simulink model "gm_soc_dlmc_rfsoc_dut"  (R2025b)
settings: Solver=FixedStepDiscrete  StartTime=0.0  StopTime=simTime  RelTol=1e-3
PreLoadFcn:
  | addpath('E:\AMC_Projects\deployModule\AMCMatlab\hdl_prj\hdlsrc\soc_dlmc_rfsoc_zcu111');
InitFcn:
  | soc_dlmc_rfsoc_init
undefined symbols (not defined in the file or in its folder): Fo, FPGAClkRate, Fs, mcTestData8PSK, mcTestDataB_FM, mcTestDataBPSK, mcTestDataCPFSK, mcTestDataDSB_AM, mcTestDataGFSK, mcTestDataPAM4, mcTestDataQAM16, mcTestDataQAM64, mcTestDataQPSK, mcTestDataSSB_AM, N, sampleTimeDL
libraries: hdlsllib x15, hdlmdlgenlib x9, simulink x2, simulink_need_slupdate x2, dsphdlsigops2 x1
CloseFcn:
  | addpath('E:\AMC_Projects\deployModule\AMCMatlab\hdl_prj\hdlsrc\soc_dlmc_rfsoc_zcu111');
  | rmpath('E:\AMC_Projects\deployModule\AMCMatlab\hdl_prj\hdlsrc\soc_dlmc_rfsoc_zcu111');
settings Model: Creator=The MathWorks, Inc.  LastModifiedBy=admin
settings SolverCC: AlgebraicLoopSolver=TrustRegion  PositivePriorityOrder=on  MaxZcPerStep=1.0
settings DataIOCC: SaveOutput=off  SaveTime=off
settings OptimizationCC: BlockReduction=off  ConditionallyExecuteInputs=off  DefaultParameterBehavior=Inlined  InheritOutputTypeSmallerThanSingle=on  EnhancedBackFolding=on  PassReuseOutputArgsAs=Individual arguments  ZeroExternalMemoryAtStartup=off  ZeroInternalMemoryAtStartup=off  MaxStackSize=64  OptimizeBlockOrder=speed  DifferentSizesBufferReuse=on  OptimizationCustomize=off  EfficientTunableParamExpr=on
settings DebuggingCC: AlgebraicLoopMsg=error  InheritedTsInSrcMsg=none  SingleTaskRateTransMsg=error  ParameterOverflowMsg=none  ParameterPrecisionLossMsg=none  ParameterTunabilityLossMsg=error  UnconnectedInputMsg=warning  SubsystemReferenceDiagnosticForUnitTest=warning  SymbolicDimsDataTypeCodeGenerationDiagnostic=none
settings HardwareCC: ProdBitPerPointer=32.0  ProdBitPerSizeT=32.0  ProdBitPerPtrDiffT=32.0  ProdLargestAtomicFloat=None  ProdIntDivRoundTo=Undefined  ProdEndianess=Unspecified  ProdWordSize=32.0  ProdHWDeviceType=ASIC/FPGA->ASIC/FPGA  TargetBitPerPointer=64.0  TargetBitPerSizeT=64.0  TargetBitPerPtrDiffT=64.0  TargetLongLongMode=on  TargetIntDivRoundTo=Zero  TargetEndianess=LittleEndian  TargetWordSize=64.0  TargetHWDeviceType=Custom Processor->MATLAB Host Computer  ProdEqTarget=off  HardwareBoardFeatureSet=SoCBlockset
settings ModelReferenceCC: EnableRefExpFcnMdlSchedulingChecks=on  ModelReferenceNumInstancesAllowed=Single
settings RTWCC: SystemTargetFile=ert.tlc  HardwareBoard=Xilinx Zynq UltraScale+ RFSoC ZCU111 Evaluation Kit  TLCOptions="-aInlineSetEventsForThisBaseRateFcn=TLC_FALSE -aSuppressMultiTaskScheduler=TLC_FALSE  -aRateBasedStepFcn=0"  TemplateMakefile=ert_default_tmf  Toolchain=Linaro AArch64 Linux v6.3.1  GPUComputeCapability=3.5  DLArmComputeVersion=19.05  Description=Embedded Coder
settings CodeAppCC: ForceParamTrailComments=on  IgnoreCustomStorageClasses=off  OperatorAnnotations=on  SimulinkDataObjDesc=on  SFDataObjDesc=on  InsertBlockDesc=on
settings ERTTargetCC: SubcomponentCodeInterfacePackaging=Nonreusable function

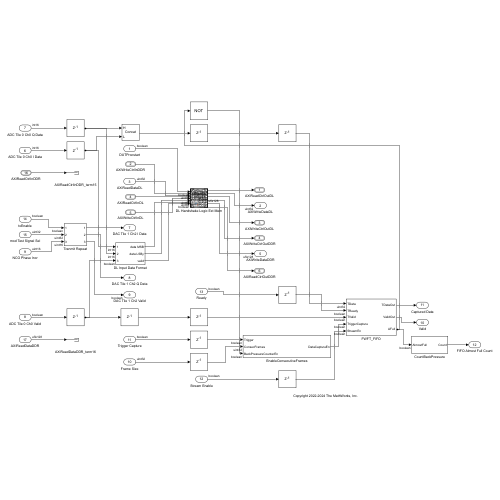
[thumbnail: Simulink's stored preview of the top-level diagram]
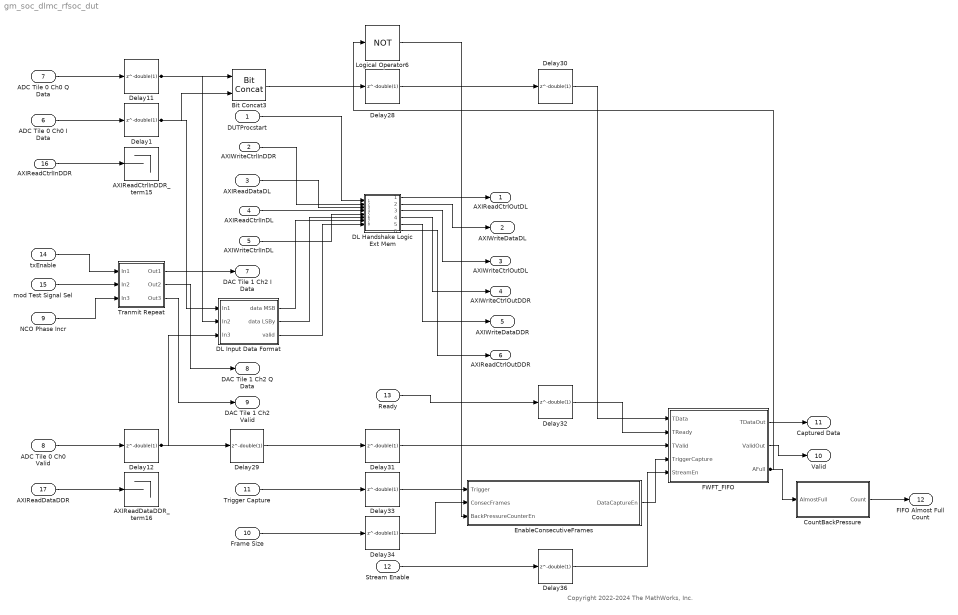
== system gm_soc_dlmc_rfsoc_dut ==
  note: Copyright 2022-2024 The MathWorks, Inc.
  DUTProcstart : Inport  OutDataTypeStr=boolean  PortDimensions=1  SampleTime=3.90625e-09
  AXIWriteCtrlInDDR : Inport  Port=2  OutDataTypeStr=Bus: BusAXIWriteCtrlS2M  SampleTime=sampleTimeDL
  AXIReadDataDL : Inport  Port=3  OutDataTypeStr=uint32  PortDimensions=1  SampleTime=3.90625e-09
  AXIReadCtrlInDL : Inport  Port=4  OutDataTypeStr=Bus: BusAXIReadCtrlS2M  SampleTime=sampleTimeDL
  AXIWriteCtrlInDL : Inport  Port=5  OutDataTypeStr=Bus: BusAXIWriteCtrlS2M  SampleTime=sampleTimeDL
  ADC Tile 0 Ch0 I Data : Inport  Port=6  OutDataTypeStr=int16  PortDimensions=1  SampleTime=3.90625e-09
  ADC Tile 0 Ch0 Q Data : Inport  Port=7  OutDataTypeStr=int16  PortDimensions=1  SampleTime=3.90625e-09
  ADC Tile 0 Ch0 Valid : Inport  Port=8  OutDataTypeStr=boolean  PortDimensions=1  SampleTime=3.90625e-09
  NCO Phase Incr : Inport  Port=9  OutDataTypeStr=uint16  PortDimensions=1  SampleTime=3.90625e-09
  Frame Size : Inport  Port=10  OutDataTypeStr=uint32  PortDimensions=1  SampleTime=3.90625e-09
  Trigger Capture : Inport  Port=11  OutDataTypeStr=boolean  PortDimensions=1  SampleTime=3.90625e-09
  Stream Enable : Inport  Port=12  OutDataTypeStr=boolean  PortDimensions=1  SampleTime=3.90625e-09
  Ready : Inport  Port=13  OutDataTypeStr=boolean  PortDimensions=1  SampleTime=3.90625e-09
  txEnable : Inport  Port=14  OutDataTypeStr=boolean  PortDimensions=1  SampleTime=3.90625e-09
  mod Test Signal Sel : Inport  Port=15  OutDataTypeStr=uint32  PortDimensions=1  SampleTime=3.90625e-09
  AXIReadCtrlInDDR : Inport  Port=16  OutDataTypeStr=Bus: BusAXIReadCtrlS2M
  AXIReadDataDDR : Inport  Port=17  OutDataTypeStr=fixdt(0, 128, 0)  PortDimensions=1  SampleTime=3.90625e-09
  AXIReadCtrlInDDR_term15 : Terminator
  AXIReadDataDDR_term16 : Terminator
  Bit Concat3 : hdlsllib/Logic and Bit Operations/Bit Concat  numInputs=2
  CountBackPressure : Subsystem
  DL Handshake Logic Ext Mem : ModelReference  ModelNameDialog=gm_soc_dlmc_handshake_ddr  SimulationMode=Normal  ModelReferenceVersion=8.1
  DL Input Data Format : Subsystem
  Delay{1,11..12,28..34,36} (11 alike) : Delay  DelayLength=double(1)  InitialCondition=0  SampleTime=3.90625e-09
  EnableConsecutiveFrames : Subsystem
  FWFT_FIFO : Subsystem
  Logical Operator6 : Logic  Operator=NOT  Inputs=1  AllPortsSameDT=off  OutDataTypeStr=boolean  SampleTime=3.90625e-09
  Tranmit Repeat : Subsystem
  AXIReadCtrlOutDL : Outport  OutDataTypeStr=Bus: BusAXIReadCtrlM2S  SampleTime=sampleTimeDL
  AXIWriteDataDL : Outport  Port=2  OutDataTypeStr=uint32  SampleTime=3.90625e-09
  AXIWriteCtrlOutDL : Outport  Port=3  OutDataTypeStr=Bus: BusAXIWriteCtrlM2S  SampleTime=sampleTimeDL
  AXIWriteCtrlOutDDR : Outport  Port=4  OutDataTypeStr=Bus:BusAXIWriteCtrlM2S  SampleTime=sampleTimeDL
  AXIWriteDataDDR : Outport  Port=5  OutDataTypeStr=fixdt(0,4*bitWidth,0)  SampleTime=3.90625e-09
  AXIReadCtrlOutDDR : Outport  Port=6  OutDataTypeStr=Bus: BusAXIReadCtrlM2S  VectorParamsAs1DForOutWhenUnconnected=off
  DAC Tile 1 Ch2 I Data : Outport  Port=7  SampleTime=3.90625e-09
  DAC Tile 1 Ch2 Q Data : Outport  Port=8  SampleTime=3.90625e-09
  DAC Tile 1 Ch2 Valid : Outport  Port=9  OutDataTypeStr=boolean  SampleTime=3.90625e-09
  Valid : Outport  Port=10  SampleTime=3.90625e-09  VectorParamsAs1DForOutWhenUnconnected=off
  Captured Data : Outport  Port=11  SampleTime=3.90625e-09  VectorParamsAs1DForOutWhenUnconnected=off
  FIFO Almost Full Count : Outport  Port=12  PortDimensions=1  SampleTime=3.90625e-09  VectorParamsAs1DForOutWhenUnconnected=off
  wires:
  Ready/1 -> Delay32/1
  Trigger Capture/1 -> Delay33/1
  ADC Tile 0 Ch0 I Data/1 -> Delay1/1
  mod Test Signal Sel/1 -> Tranmit Repeat/2(In2)
  ADC Tile 0 Ch0 Valid/1 -> Delay12/1
  AXIReadDataDDR/1 -> AXIReadDataDDR_term16/1
  Stream Enable/1 -> Delay36/1
  AXIWriteCtrlInDL/1 -> DL Handshake Logic Ext Mem/5
  ADC Tile 0 Ch0 Q Data/1 -> Delay11/1
  AXIReadCtrlInDDR/1 -> AXIReadCtrlInDDR_term15/1
  txEnable/1 -> Tranmit Repeat/1(In1)
  NCO Phase Incr/1 -> Tranmit Repeat/3(In3)
  Delay11/1 -> Bit Concat3/1, DL Input Data Format/2(In2)
  Delay1/1 -> Bit Concat3/2, DL Input Data Format/1(In1)
  Tranmit Repeat/1(Out1) -> DAC Tile 1 Ch2 I Data/1
  Delay28/1 -> Delay30/1
  Tranmit Repeat/2(Out2) -> DAC Tile 1 Ch2 Q Data/1
  Tranmit Repeat/3(Out3) -> DAC Tile 1 Ch2 Valid/1
  Delay12/1 -> Delay29/1, DL Input Data Format/3(In3)
  Bit Concat3/1 -> Delay28/1
  AXIReadDataDL/1 -> DL Handshake Logic Ext Mem/3
  DUTProcstart/1 -> DL Handshake Logic Ext Mem/1
  AXIWriteCtrlInDDR/1 -> DL Handshake Logic Ext Mem/2
  AXIReadCtrlInDL/1 -> DL Handshake Logic Ext Mem/4
  DL Input Data Format/1(data MSB) -> DL Handshake Logic Ext Mem/7
  Delay31/1 -> FWFT_FIFO/3(TValid)
  DL Input Data Format/2(data LSBy) -> DL Handshake Logic Ext Mem/6
  DL Input Data Format/3(valid) -> DL Handshake Logic Ext Mem/8
  Delay29/1 -> Delay31/1
  Frame Size/1 -> Delay34/1
  EnableConsecutiveFrames/1(DataCaptureEn) -> FWFT_FIFO/4(TriggerCapture)
  Logical Operator6/1 -> EnableConsecutiveFrames/3(BackPressureCounterEn)
  DL Handshake Logic Ext Mem/5 -> AXIWriteDataDDR/1
  DL Handshake Logic Ext Mem/1 -> AXIReadCtrlOutDL/1
  Delay30/1 -> FWFT_FIFO/1(TData)
  DL Handshake Logic Ext Mem/6 -> AXIReadCtrlOutDDR/1
  DL Handshake Logic Ext Mem/2 -> AXIWriteDataDL/1
  DL Handshake Logic Ext Mem/3 -> AXIWriteCtrlOutDL/1
  DL Handshake Logic Ext Mem/4 -> AXIWriteCtrlOutDDR/1
  FWFT_FIFO/3(AFull) -> Logical Operator6/1, CountBackPressure/1(AlmostFull)
  Delay33/1 -> EnableConsecutiveFrames/1(Trigger)
  Delay34/1 -> EnableConsecutiveFrames/2(ConsecFrames)
  FWFT_FIFO/2(ValidOut) -> Valid/1
  Delay32/1 -> FWFT_FIFO/2(TReady)
  CountBackPressure/1(Count) -> FIFO Almost Full Count/1
  FWFT_FIFO/1(TDataOut) -> Captured Data/1
  Delay36/1 -> FWFT_FIFO/5(StreamEn)

== system gm_soc_dlmc_rfsoc_dut/CountBackPressure ==
  AlmostFull : Inport  OutDataTypeStr=boolean  PortDimensions=1  SampleTime=3.90625e-09
  Add : Sum  OutDataTypeStr=uint32  AccumDataTypeStr=uint32  SampleTime=3.90625e-09
  Data Type Conversion : DataTypeConversion  OutDataTypeStr=uint32  SampleTime=3.90625e-09  SaturateOnIntegerOverflow=off  RndMeth=Floor
  Delay16 : Delay  DelayLength=double(1)  InitialCondition=0  SampleTime=3.90625e-09
  Count : Outport  SampleTime=3.90625e-09  VectorParamsAs1DForOutWhenUnconnected=off
  wires:
  Data Type Conversion/1 -> Add/1
  AlmostFull/1 -> Data Type Conversion/1
  Add/1 -> Delay16/1
  Delay16/1 -> Add/2, Count/1

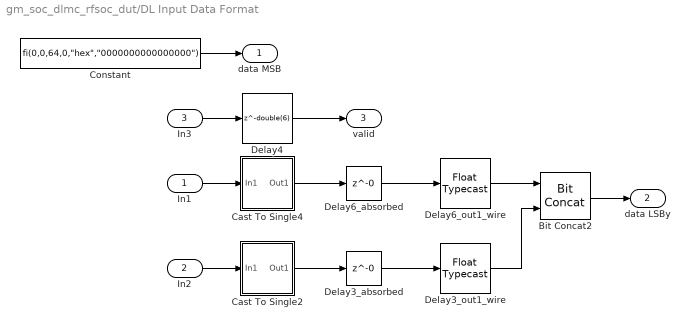
== system gm_soc_dlmc_rfsoc_dut/DL Input Data Format ==
  In1 : Inport  OutDataTypeStr=int16  PortDimensions=1  SampleTime=3.90625e-09
  In2 : Inport  Port=2  OutDataTypeStr=int16  PortDimensions=1  SampleTime=3.90625e-09
  In3 : Inport  Port=3  OutDataTypeStr=boolean  PortDimensions=1  SampleTime=3.90625e-09
  Bit Concat2 : hdlsllib/Logic and Bit Operations/Bit Concat  numInputs=2
  Cast To Single2 : Subsystem
      mask Display: disp('NFP\nconv');
  Cast To Single4 : Subsystem
      mask Display: disp('NFP\nconv');
  Constant : Constant  Value="fi(0,0,64,0,\"hex\",\"0000000000000000\")"  OutDataTypeStr=fixdt(0, 64, 0)  SampleTime=3.90625e-09
  Delay3_absorbed : Delay  DelayLength=0
  Delay3_out1_wire : FloatTypecast
  Delay4 : Delay  DelayLength=double(6)  InitialCondition=0  SampleTime=3.90625e-09
  Delay6_absorbed : Delay  DelayLength=0
  Delay6_out1_wire : FloatTypecast
  data MSB : Outport  SampleTime=3.90625e-09
  data LSBy : Outport  Port=2  SampleTime=3.90625e-09
  valid : Outport  Port=3  SampleTime=3.90625e-09
  wires:
  Delay6_absorbed/1 -> Delay6_out1_wire/1
  In2/1 -> Cast To Single2/1(In1)
  Constant/1 -> data MSB/1
  In3/1 -> Delay4/1
  Cast To Single4/1(Out1) -> Delay6_absorbed/1
  In1/1 -> Cast To Single4/1(In1)
  Delay4/1 -> valid/1
  Cast To Single2/1(Out1) -> Delay3_absorbed/1
  Delay3_absorbed/1 -> Delay3_out1_wire/1
  Delay6_out1_wire/1 -> Bit Concat2/1
  Delay3_out1_wire/1 -> Bit Concat2/2
  Bit Concat2/1 -> data LSBy/1

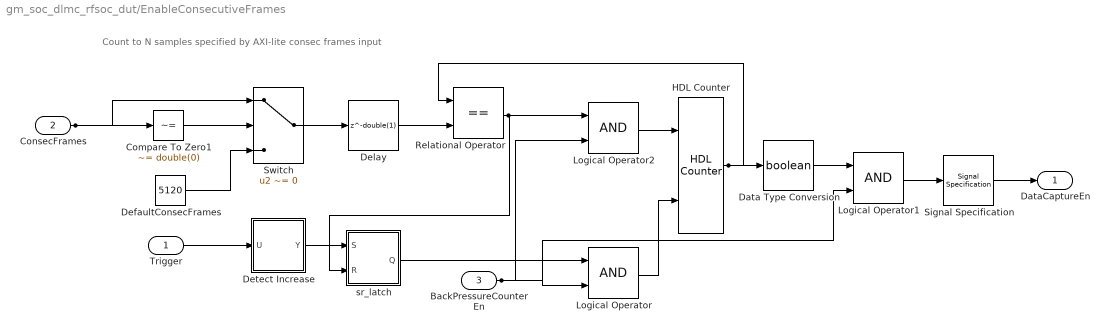
== system gm_soc_dlmc_rfsoc_dut/EnableConsecutiveFrames ==
  note: Count to N samples specified by AXI-lite consec frames input
  Trigger : Inport  OutDataTypeStr=boolean  PortDimensions=1  SampleTime=3.90625e-09
  ConsecFrames : Inport  Port=2  OutDataTypeStr=uint32  PortDimensions=1  SampleTime=3.90625e-09
  BackPressureCounterEn : Inport  Port=3  OutDataTypeStr=boolean  PortDimensions=1  SampleTime=3.90625e-09
  Compare To Zero1 : simulink/Logic and Bit Operations/Compare To Constant  relop=~=  const=double(0)  OutDataTypeStr=boolean
  Data Type Conversion : DataTypeConversion  OutDataTypeStr=boolean  SampleTime=3.90625e-09  SaturateOnIntegerOverflow=off  RndMeth=Floor
  DefaultConsecFrames : Constant  Value=5120  OutDataTypeStr=uint32  SampleTime=3.90625e-09
  Delay : Delay  DelayLength=double(1)  InitialCondition=0  SampleTime=3.90625e-09
  Detect Increase : Subsystem  mask(Detect Increase){vinit=double(0), InputProcessing=Elements as channels (sample based), OutDataTypeStr=boolean}
      mask prompts: vinit "Simulink:masks:InitialCondition_MP"; InputProcessing "Simulink:masks:InputProcessing_MP"; OutDataTypeStr "Simulink:masks:OutputDataType_MP"
      mask help: Simulink:masks:DetectIncrease_MD
      mask init:
      | InputProcessing = 'Elements as channels (sample based)';
      | OutDataTypeStr = 'boolean';
      | vinit = double(0);
      mask TypeOptions InputProcessing: Simulink:masks:ColumnsAsChannelsFrameBased | Simulink:masks:ElementsAsChannelsSampleBased
      mask TypeOptions OutDataTypeStr: Simulink:masks:uint8 | Simulink:masks:boolean
      mask Display: fprintf('U > U/z')
  HDL Counter : hdlsllib/Sources/HDL Counter  CountType=Free running  CountInit=0  CountStep=1  CountMax=25  CountFromType=Initial value  CountFrom=0  CountResetPort=on  CountLoadPort=off  CountEnbPort=on  CountDirPort=off  CountHitOutputPort=off  CountDataType=Unsigned  CountWordLen=32  CountFracLen=0  CountSampTime=1
  Logical Operator : Logic  AllPortsSameDT=off  OutDataTypeStr=boolean  SampleTime=3.90625e-09
  Logical Operator1 : Logic  AllPortsSameDT=off  OutDataTypeStr=boolean  SampleTime=3.90625e-09
  Logical Operator2 : Logic  AllPortsSameDT=off  OutDataTypeStr=boolean  SampleTime=3.90625e-09
  Relational Operator : RelationalOperator  Operator===  OutDataTypeStr=boolean  SampleTime=3.90625e-09  InputSameDT=off
  Signal Specification : SignalSpecification  OutDataTypeStr=boolean  Dimensions=1
  Switch : Switch  Criteria=u2 ~= 0  Threshold="fi(0,0,1,0,\"hex\",\"0\")"  OutDataTypeStr=uint32  SampleTime=3.90625e-09  SaturateOnIntegerOverflow=off  InputSameDT=off
  sr_latch : Subsystem
  DataCaptureEn : Outport  SampleTime=3.90625e-09  VectorParamsAs1DForOutWhenUnconnected=off
  wires:
  Trigger/1 -> Detect Increase/1(U)
  ConsecFrames/1 -> Switch/1, Compare To Zero1/1
  Compare To Zero1/1 -> Switch/2
  Signal Specification/1 -> DataCaptureEn/1
  Delay/1 -> Relational Operator/2
  Relational Operator/1 -> sr_latch/2(R), Logical Operator2/1
  DefaultConsecFrames/1 -> Switch/3
  Logical Operator/1 -> HDL Counter/2
  Switch/1 -> Delay/1
  Detect Increase/1(Y) -> sr_latch/1(S)
  sr_latch/1(Q) -> Logical Operator/1
  BackPressureCounterEn/1 -> Logical Operator1/2, Logical Operator2/2, Logical Operator/2
  Logical Operator2/1 -> HDL Counter/1
  HDL Counter/1 -> Data Type Conversion/1, Relational Operator/1
  Data Type Conversion/1 -> Logical Operator1/1
  Logical Operator1/1 -> Signal Specification/1

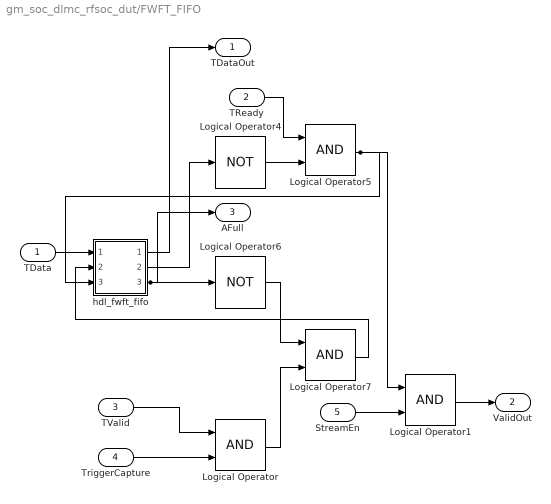
== system gm_soc_dlmc_rfsoc_dut/FWFT_FIFO ==
  TData : Inport  OutDataTypeStr=uint32  PortDimensions=1  SampleTime=3.90625e-09
  TReady : Inport  Port=2  OutDataTypeStr=boolean  PortDimensions=1  SampleTime=3.90625e-09
  TValid : Inport  Port=3  OutDataTypeStr=boolean  PortDimensions=1  SampleTime=3.90625e-09
  TriggerCapture : Inport  Port=4  OutDataTypeStr=boolean  PortDimensions=1  SampleTime=3.90625e-09
  StreamEn : Inport  Port=5  OutDataTypeStr=boolean  PortDimensions=1  SampleTime=3.90625e-09
  Logical Operator{,1,5,7} (4 alike) : Logic  AllPortsSameDT=off  OutDataTypeStr=boolean  SampleTime=3.90625e-09
  Logical Operator4 : Logic  Operator=NOT  Inputs=1  AllPortsSameDT=off  OutDataTypeStr=boolean  SampleTime=3.90625e-09
  Logical Operator6 : Logic  Operator=NOT  Inputs=1  AllPortsSameDT=off  OutDataTypeStr=boolean  SampleTime=3.90625e-09
  hdl_fwft_fifo : Subsystem  mask{FIFO_DEPTH=double(10240), AFULL_THRESH=double(10)}
      mask prompts: FIFO_DEPTH "FIFO Depth"; AFULL_THRESH "Almost Full Threshold"
      mask init:
      | AFULL_THRESH = double(10);
      | FIFO_CNT_BITS = double(14);
      | FIFO_DEPTH = double(10240);
  TDataOut : Outport  SampleTime=3.90625e-09  VectorParamsAs1DForOutWhenUnconnected=off
  ValidOut : Outport  Port=2  SampleTime=3.90625e-09  VectorParamsAs1DForOutWhenUnconnected=off
  AFull : Outport  Port=3  SampleTime=3.90625e-09  VectorParamsAs1DForOutWhenUnconnected=off
  wires:
  TriggerCapture/1 -> Logical Operator/2
  StreamEn/1 -> Logical Operator1/2
  TData/1 -> hdl_fwft_fifo/1(data_i)
  hdl_fwft_fifo/1(data_o) -> TDataOut/1
  Logical Operator4/1 -> Logical Operator5/2
  hdl_fwft_fifo/3(afull) -> AFull/1, Logical Operator6/1
  hdl_fwft_fifo/2(empty_o) -> Logical Operator4/1
  TReady/1 -> Logical Operator5/1
  TValid/1 -> Logical Operator/1
  Logical Operator1/1 -> ValidOut/1
  Logical Operator/1 -> Logical Operator7/2
  Logical Operator6/1 -> Logical Operator7/1
  Logical Operator5/1 -> hdl_fwft_fifo/3(rd_ack), Logical Operator1/1
  Logical Operator7/1 -> hdl_fwft_fifo/2(push)

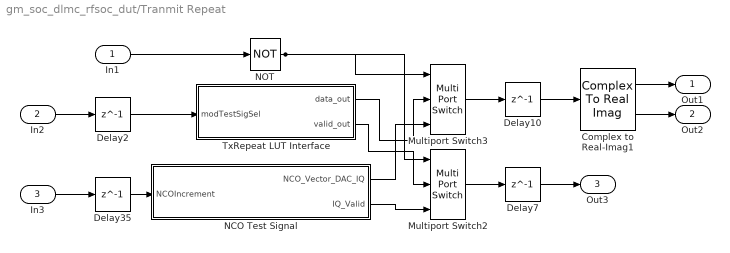
== system gm_soc_dlmc_rfsoc_dut/Tranmit Repeat ==
  In1 : Inport  OutDataTypeStr=boolean  PortDimensions=1  SampleTime=3.90625e-09
  In2 : Inport  Port=2  OutDataTypeStr=uint32  PortDimensions=1  SampleTime=3.90625e-09
  In3 : Inport  Port=3  OutDataTypeStr=uint16  PortDimensions=1  SampleTime=3.90625e-09
  Complex to Real-Imag1 : ComplexToRealImag
  Delay{2,7,10,35} (4 alike) : Delay  DelayLength=1
  Multiport Switch2 : MultiPortSwitch  DataPortOrder=Zero-based contiguous  Inputs=2  zeroidx=on  SaturateOnIntegerOverflow=off  InputSameDT=off
  Multiport Switch3 : MultiPortSwitch  DataPortOrder=Zero-based contiguous  Inputs=2  zeroidx=on  OutDataTypeStr=int16  SaturateOnIntegerOverflow=off  InputSameDT=off
  NCO Test Signal : Subsystem
  NOT : Logic  Operator=NOT  IconShape=distinctive  AllPortsSameDT=off  OutDataTypeStr=boolean
  TxRepeat LUT Interface : Subsystem
  Out1 : Outport  SampleTime=3.90625e-09
  Out2 : Outport  Port=2  SampleTime=3.90625e-09
  Out3 : Outport  Port=3  SampleTime=3.90625e-09
  wires:
  In1/1 -> NOT/1
  In2/1 -> Delay2/1
  NOT/1 -> Multiport Switch3/1, Multiport Switch2/1
  In3/1 -> Delay35/1
  TxRepeat LUT Interface/2(valid_out) -> Multiport Switch2/2
  Delay35/1 -> NCO Test Signal/1(NCOIncrement)
  Delay2/1 -> TxRepeat LUT Interface/1(modTestSigSel)
  TxRepeat LUT Interface/1(data_out) -> Multiport Switch3/2
  NCO Test Signal/1(NCO_Vector_DAC_IQ) -> Multiport Switch3/3
  NCO Test Signal/2(IQ_Valid) -> Multiport Switch2/3
  Multiport Switch3/1 -> Delay10/1
  Multiport Switch2/1 -> Delay7/1
  Delay10/1 -> Complex to Real-Imag1/1
  Complex to Real-Imag1/2 -> Out2/1
  Delay7/1 -> Out3/1
  Complex to Real-Imag1/1 -> Out1/1

== system gm_soc_dlmc_rfsoc_dut/DL Input Data Format/Cast To Single2 ==
  In1 : Inport
  Cast To Single2 : DataTypeConversion  OutDataTypeStr=single  SampleTime=3.90625e-09  SaturateOnIntegerOverflow=off  RndMeth=Floor
  Cast To Single2_pd1 : Delay  DelayLength=6
  Out1 : Outport
  wires:
  In1/1 -> Cast To Single2/1
  Cast To Single2/1 -> Cast To Single2_pd1/1
  Cast To Single2_pd1/1 -> Out1/1

== system gm_soc_dlmc_rfsoc_dut/DL Input Data Format/Cast To Single4 ==
  In1 : Inport
  Cast To Single4 : DataTypeConversion  OutDataTypeStr=single  SampleTime=3.90625e-09  SaturateOnIntegerOverflow=off  RndMeth=Floor
  Cast To Single4_pd1 : Delay  DelayLength=6
  Out1 : Outport
  wires:
  In1/1 -> Cast To Single4/1
  Cast To Single4/1 -> Cast To Single4_pd1/1
  Cast To Single4_pd1/1 -> Out1/1

== system gm_soc_dlmc_rfsoc_dut/EnableConsecutiveFrames/Detect Increase ==
  note: U(k)
  note: Edge
  U : Inport  OutDataTypeStr=boolean  SampleTime=3.90625e-09
  Delay Input1 : UnitDelay  Description=Store in Global RAM  DisableCoverage=on  InitialCondition=vinit  SampleTime=-1  HasFrameUpgradeWarning=on
  FixPt Relational Operator : RelationalOperator  Operator=>  OutDataTypeStr=boolean  ZeroCross=off  InputSameDT=off
  Y : Outport  SampleTime=3.90625e-09  InitialOutput=0
  wires:
  FixPt Relational Operator/1 -> Y/1
  Delay Input1/1 -> FixPt Relational Operator/2
  U/1 -> FixPt Relational Operator/1, Delay Input1/1

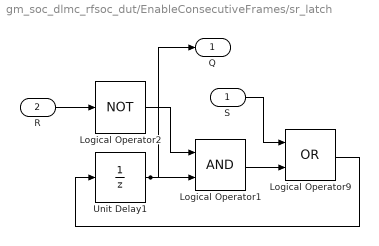
== system gm_soc_dlmc_rfsoc_dut/EnableConsecutiveFrames/sr_latch ==
  S : Inport  OutDataTypeStr=boolean  PortDimensions=1  SampleTime=3.90625e-09
  R : Inport  Port=2  OutDataTypeStr=boolean  PortDimensions=1  SampleTime=3.90625e-09
  Logical Operator1 : Logic  AllPortsSameDT=off  OutDataTypeStr=boolean  SampleTime=3.90625e-09
  Logical Operator2 : Logic  Operator=NOT  Inputs=1  AllPortsSameDT=off  OutDataTypeStr=boolean  SampleTime=3.90625e-09
  Logical Operator9 : Logic  Operator=OR  AllPortsSameDT=off  OutDataTypeStr=boolean  SampleTime=3.90625e-09
  Unit Delay1 : UnitDelay  SampleTime=3.90625e-09
  Q : Outport  SampleTime=3.90625e-09  VectorParamsAs1DForOutWhenUnconnected=off
  wires:
  Logical Operator1/1 -> Logical Operator9/2
  Logical Operator2/1 -> Logical Operator1/1
  R/1 -> Logical Operator2/1
  Logical Operator9/1 -> Unit Delay1/1
  Unit Delay1/1 -> Q/1, Logical Operator1/2
  S/1 -> Logical Operator9/1

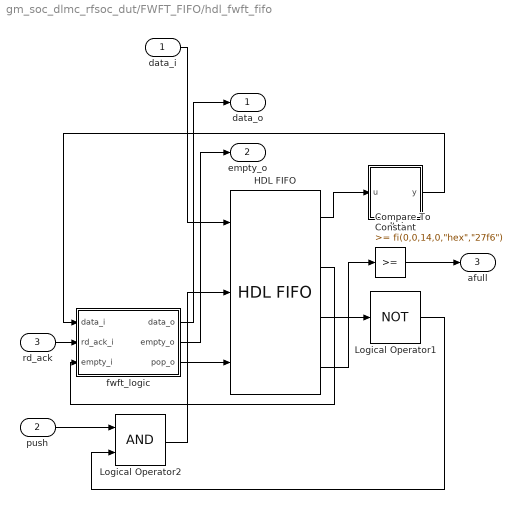
== system gm_soc_dlmc_rfsoc_dut/FWFT_FIFO/hdl_fwft_fifo ==
  data_i : Inport  OutDataTypeStr=uint32  PortDimensions=1  SampleTime=3.90625e-09
  push : Inport  Port=2  OutDataTypeStr=boolean  PortDimensions=1  SampleTime=3.90625e-09
  rd_ack : Inport  Port=3  OutDataTypeStr=boolean  PortDimensions=1  SampleTime=3.90625e-09
  Compare To Constant : simulink/Logic and Bit Operations/Compare To Constant  relop=>=  const="fi(0,0,14,0,\"hex\",\"27f6\")"  OutDataTypeStr=boolean
  HDL FIFO : hdlsllib/HDL RAMs/HDL FIFO  fifo_size=FIFO_DEPTH  mode=Classic  ratio=1  push_msg=Error  pop_msg=Ignore  show_empty=on  show_full=on  show_num=on  LabelModeActiveChoice_Mode=Classic  rst_port=off
  Logical Operator1 : Logic  Operator=NOT  Inputs=1  AllPortsSameDT=off  OutDataTypeStr=boolean  SampleTime=3.90625e-09
  Logical Operator2 : Logic  AllPortsSameDT=off  OutDataTypeStr=boolean  SampleTime=3.90625e-09
  dtci : Subsystem  mask(Conversion Inherited){ConvertRealWorld=Real World Value, RndMeth=Floor, DoSatur=off}
      mask prompts: ConvertRealWorld "Simulink:masks:InputAndOutputToHaveEqual_MP"; RndMeth "Simulink:masks:IntegerRoundingMode_MP"; DoSatur "Simulink:masks:SaturateToMaxOrMinWhenOverflowsOccur_MP"
      mask help: Simulink:masks:ConversionInherited_MD
      mask init:
      | ConvertRealWorld = double(1);
      | DoSatur = double(0);
      | RndMeth = double(3);
      mask TypeOptions ConvertRealWorld: Simulink:masks:RealWorldValue | Simulink:masks:StoredInteger
      mask TypeOptions RndMeth: Simulink:masks:Ceiling | Simulink:masks:Convergent | Simulink:masks:Floor | Simulink:masks:Nearest | Simulink:masks:Round | Simulink:masks:Simplest | Simulink:masks:Zero
      mask Display:
      | port_label('Input',2,'u');
      | port_label('Output',1,'y');
      |     if(get_param(gcbh,'ConvertRealWorld') == "Stored Integer")
      |        disp('SI')
      |     else
      |        disp('Convert')
      |     end
  fwft_logic : Subsystem
  data_o : Outport  SampleTime=3.90625e-09  VectorParamsAs1DForOutWhenUnconnected=off
  empty_o : Outport  Port=2  SampleTime=3.90625e-09  VectorParamsAs1DForOutWhenUnconnected=off
  afull : Outport  Port=3  SampleTime=3.90625e-09  VectorParamsAs1DForOutWhenUnconnected=off
  wires:
  HDL FIFO/1 -> dtci/1(u)
  data_i/1 -> HDL FIFO/1
  push/1 -> Logical Operator2/1
  rd_ack/1 -> fwft_logic/2(rd_ack_i)
  fwft_logic/2(empty_o) -> empty_o/1
  fwft_logic/1(data_o) -> data_o/1
  Logical Operator2/1 -> HDL FIFO/2
  fwft_logic/3(pop_o) -> HDL FIFO/3
  HDL FIFO/2 -> fwft_logic/3(empty_i)
  HDL FIFO/3 -> Logical Operator1/1
  HDL FIFO/4 -> Compare To Constant/1
  dtci/1(y) -> fwft_logic/1(data_i)
  Compare To Constant/1 -> afull/1
  Logical Operator1/1 -> Logical Operator2/2

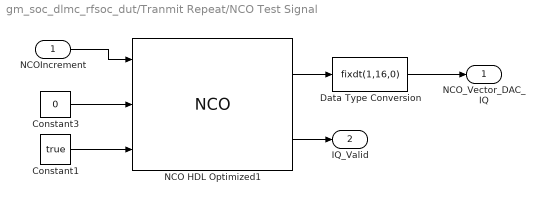
== system gm_soc_dlmc_rfsoc_dut/Tranmit Repeat/NCO Test Signal ==
  NCOIncrement : Inport  OutDataTypeStr=uint16  PortDimensions=1  SampleTime=3.90625e-09
  Constant1 : Constant  Value=true  OutDataTypeStr=boolean  SampleTime=-1
  Constant3 : Constant  Value=0  OutDataTypeStr=uint16  SampleTime=-1
  Data Type Conversion : DataTypeConversion  OutDataTypeStr=fixdt(1,16,0)  ConvertRealWorld=Stored Integer (SI)  SaturateOnIntegerOverflow=off  RndMeth=Floor
  NCO HDL Optimized1 : dsphdlsigops2/NCO  PhaseIncrementSource=Input port  PhaseIncrement=round(Fo*(2^N)/Fs)  PhaseOffsetSource=Input port  PhaseOffset=0  DitherSource=Property  NumDitherBits=4  SamplesPerFrame=1  LUTCompress=on  ResetAction=off  Waveform=Complex exponential  PhasePort=off  SimulateUsing=Code generation  AccumulatorWL=14  PhaseQuantization=off  NumQuantizerAccumulatorBits=12  OutputDataType=Binary point scaling  OutputWL=14  OutputFL=12
  NCO_Vector_DAC_IQ : Outport  SampleTime=3.90625e-09  VectorParamsAs1DForOutWhenUnconnected=off
  IQ_Valid : Outport  Port=2  SampleTime=3.90625e-09  VectorParamsAs1DForOutWhenUnconnected=off
  wires:
  NCOIncrement/1 -> NCO HDL Optimized1/1
  Data Type Conversion/1 -> NCO_Vector_DAC_IQ/1
  NCO HDL Optimized1/2 -> IQ_Valid/1
  NCO HDL Optimized1/1 -> Data Type Conversion/1
  Constant1/1 -> NCO HDL Optimized1/3
  Constant3/1 -> NCO HDL Optimized1/2

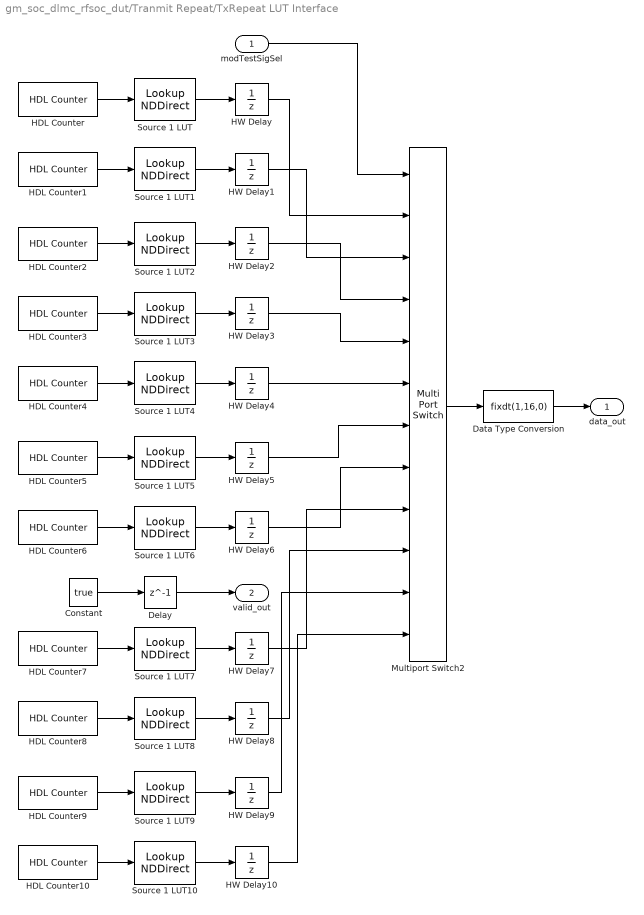
== system gm_soc_dlmc_rfsoc_dut/Tranmit Repeat/TxRepeat LUT Interface ==
  modTestSigSel : Inport  OutDataTypeStr=uint32  PortDimensions=1  SampleTime=3.90625e-09
  Constant : Constant  Value=true  OutDataTypeStr=boolean  SampleTime=-1
  Data Type Conversion : DataTypeConversion  OutDataTypeStr=fixdt(1,16,0)  ConvertRealWorld=Stored Integer (SI)  SaturateOnIntegerOverflow=off  RndMeth=Floor
  Delay : Delay  DelayLength=1
  HDL Counter : hdlsllib/Sources/HDL Counter  CountType=Count limited  CountInit=0  CountStep=1  CountMax=length(mcTestDataQAM16)-1  CountFromType=Initial value  CountFrom=0  CountResetPort=off  CountLoadPort=off  CountEnbPort=off  CountDirPort=off  CountHitOutputPort=off  CountDataType=Unsigned  CountWordLen=nextpow2(length(mcTestDataQAM16))  CountFracLen=0  CountSampTime=1/FPGAClkRate
  HDL Counter1 : hdlsllib/Sources/HDL Counter  CountType=Count limited  CountInit=0  CountStep=1  CountMax=length(mcTestDataQAM64)-1  CountFromType=Initial value  CountFrom=0  CountResetPort=off  CountLoadPort=off  CountEnbPort=off  CountDirPort=off  CountHitOutputPort=off  CountDataType=Unsigned  CountWordLen=nextpow2(length(mcTestDataQAM64))  CountFracLen=0  CountSampTime=1/FPGAClkRate
  HDL Counter10 : hdlsllib/Sources/HDL Counter  CountType=Count limited  CountInit=0  CountStep=1  CountMax=length(mcTestDataSSB_AM)-1  CountFromType=Initial value  CountFrom=0  CountResetPort=off  CountLoadPort=off  CountEnbPort=off  CountDirPort=off  CountHitOutputPort=off  CountDataType=Unsigned  CountWordLen=nextpow2(length(mcTestDataSSB_AM))  CountFracLen=0  CountSampTime=1/FPGAClkRate
  HDL Counter2 : hdlsllib/Sources/HDL Counter  CountType=Count limited  CountInit=0  CountStep=1  CountMax=length(mcTestData8PSK)-1  CountFromType=Initial value  CountFrom=0  CountResetPort=off  CountLoadPort=off  CountEnbPort=off  CountDirPort=off  CountHitOutputPort=off  CountDataType=Unsigned  CountWordLen=nextpow2(length(mcTestData8PSK))  CountFracLen=0  CountSampTime=1/FPGAClkRate
  HDL Counter3 : hdlsllib/Sources/HDL Counter  CountType=Count limited  CountInit=0  CountStep=1  CountMax=length(mcTestDataB_FM)-1  CountFromType=Initial value  CountFrom=0  CountResetPort=off  CountLoadPort=off  CountEnbPort=off  CountDirPort=off  CountHitOutputPort=off  CountDataType=Unsigned  CountWordLen=nextpow2(length(mcTestDataB_FM))  CountFracLen=0  CountSampTime=1/FPGAClkRate
  HDL Counter4 : hdlsllib/Sources/HDL Counter  CountType=Count limited  CountInit=0  CountStep=1  CountMax=length(mcTestDataBPSK)-1  CountFromType=Initial value  CountFrom=0  CountResetPort=off  CountLoadPort=off  CountEnbPort=off  CountDirPort=off  CountHitOutputPort=off  CountDataType=Unsigned  CountWordLen=nextpow2(length(mcTestDataBPSK))  CountFracLen=0  CountSampTime=1/FPGAClkRate
  HDL Counter5 : hdlsllib/Sources/HDL Counter  CountType=Count limited  CountInit=0  CountStep=1  CountMax=length(mcTestDataCPFSK)-1  CountFromType=Initial value  CountFrom=0  CountResetPort=off  CountLoadPort=off  CountEnbPort=off  CountDirPort=off  CountHitOutputPort=off  CountDataType=Unsigned  CountWordLen=nextpow2(length(mcTestDataCPFSK))  CountFracLen=0  CountSampTime=1/FPGAClkRate
  HDL Counter6 : hdlsllib/Sources/HDL Counter  CountType=Count limited  CountInit=0  CountStep=1  CountMax=length(mcTestDataDSB_AM)-1  CountFromType=Initial value  CountFrom=0  CountResetPort=off  CountLoadPort=off  CountEnbPort=off  CountDirPort=off  CountHitOutputPort=off  CountDataType=Unsigned  CountWordLen=nextpow2(length(mcTestDataDSB_AM))  CountFracLen=0  CountSampTime=1/FPGAClkRate
  HDL Counter7 : hdlsllib/Sources/HDL Counter  CountType=Count limited  CountInit=0  CountStep=1  CountMax=length(mcTestDataGFSK)-1  CountFromType=Initial value  CountFrom=0  CountResetPort=off  CountLoadPort=off  CountEnbPort=off  CountDirPort=off  CountHitOutputPort=off  CountDataType=Unsigned  CountWordLen=nextpow2(length(mcTestDataGFSK))  CountFracLen=0  CountSampTime=1/FPGAClkRate
  HDL Counter8 : hdlsllib/Sources/HDL Counter  CountType=Count limited  CountInit=0  CountStep=1  CountMax=length(mcTestDataPAM4)-1  CountFromType=Initial value  CountFrom=0  CountResetPort=off  CountLoadPort=off  CountEnbPort=off  CountDirPort=off  CountHitOutputPort=off  CountDataType=Unsigned  CountWordLen=nextpow2(length(mcTestDataPAM4))  CountFracLen=0  CountSampTime=1/FPGAClkRate
  HDL Counter9 : hdlsllib/Sources/HDL Counter  CountType=Count limited  CountInit=0  CountStep=1  CountMax=length(mcTestDataQPSK)-1  CountFromType=Initial value  CountFrom=0  CountResetPort=off  CountLoadPort=off  CountEnbPort=off  CountDirPort=off  CountHitOutputPort=off  CountDataType=Unsigned  CountWordLen=nextpow2(length(mcTestDataQPSK))  CountFracLen=0  CountSampTime=1/FPGAClkRate
  HW Delay{,1..10} (11 alike) : UnitDelay  SampleTime=-1  HasFrameUpgradeWarning=on
  Multiport Switch2 : MultiPortSwitch  DataPortOrder=Zero-based contiguous  Inputs=11  zeroidx=on  OutDataTypeStr=fixdt(1, 16, 14)  SaturateOnIntegerOverflow=off  InputSameDT=off
  Source 1 LUT : LookupNDDirect  NumberOfTableDimensions=1  Table=mcTestDataQAM16  DiagnosticForOutOfRangeInput=Error  TableDataTypeStr=fixdt(1,16,14)
  Source 1 LUT1 : LookupNDDirect  NumberOfTableDimensions=1  Table=mcTestDataQAM64  DiagnosticForOutOfRangeInput=Error  TableDataTypeStr=fixdt(1,16,14)
  Source 1 LUT10 : LookupNDDirect  NumberOfTableDimensions=1  Table=mcTestDataSSB_AM  DiagnosticForOutOfRangeInput=Error  TableDataTypeStr=fixdt(1,16,14)
  Source 1 LUT2 : LookupNDDirect  NumberOfTableDimensions=1  Table=mcTestData8PSK  DiagnosticForOutOfRangeInput=Error  TableDataTypeStr=fixdt(1,16,14)
  Source 1 LUT3 : LookupNDDirect  NumberOfTableDimensions=1  Table=mcTestDataB_FM  DiagnosticForOutOfRangeInput=Error  TableDataTypeStr=fixdt(1,16,14)
  Source 1 LUT4 : LookupNDDirect  NumberOfTableDimensions=1  Table=mcTestDataBPSK  DiagnosticForOutOfRangeInput=Error  TableDataTypeStr=fixdt(1,16,14)
  Source 1 LUT5 : LookupNDDirect  NumberOfTableDimensions=1  Table=mcTestDataCPFSK  DiagnosticForOutOfRangeInput=Error  TableDataTypeStr=fixdt(1,16,14)
  Source 1 LUT6 : LookupNDDirect  NumberOfTableDimensions=1  Table=mcTestDataDSB_AM  DiagnosticForOutOfRangeInput=Error  TableDataTypeStr=fixdt(1,16,14)
  Source 1 LUT7 : LookupNDDirect  NumberOfTableDimensions=1  Table=mcTestDataGFSK  DiagnosticForOutOfRangeInput=Error  TableDataTypeStr=fixdt(1,16,14)
  Source 1 LUT8 : LookupNDDirect  NumberOfTableDimensions=1  Table=mcTestDataPAM4  DiagnosticForOutOfRangeInput=Error  TableDataTypeStr=fixdt(1,16,14)
  Source 1 LUT9 : LookupNDDirect  NumberOfTableDimensions=1  Table=mcTestDataQPSK  DiagnosticForOutOfRangeInput=Error  TableDataTypeStr=fixdt(1,16,14)
  data_out : Outport  SampleTime=3.90625e-09
  valid_out : Outport  Port=2  SampleTime=3.90625e-09
  wires:
  Source 1 LUT7/1 -> HW Delay7/1
  HDL Counter6/1 -> Source 1 LUT6/1
  Source 1 LUT9/1 -> HW Delay9/1
  HDL Counter/1 -> Source 1 LUT/1
  HDL Counter1/1 -> Source 1 LUT1/1
  HDL Counter5/1 -> Source 1 LUT5/1
  HDL Counter2/1 -> Source 1 LUT2/1
  Source 1 LUT6/1 -> HW Delay6/1
  Source 1 LUT2/1 -> HW Delay2/1
  HDL Counter3/1 -> Source 1 LUT3/1
  HW Delay10/1 -> Multiport Switch2/12
  Constant/1 -> Delay/1
  HW Delay1/1 -> Multiport Switch2/3
  HDL Counter4/1 -> Source 1 LUT4/1
  HDL Counter7/1 -> Source 1 LUT7/1
  HDL Counter10/1 -> Source 1 LUT10/1
  HDL Counter8/1 -> Source 1 LUT8/1
  HW Delay8/1 -> Multiport Switch2/10
  Source 1 LUT10/1 -> HW Delay10/1
  HDL Counter9/1 -> Source 1 LUT9/1
  Source 1 LUT/1 -> HW Delay/1
  Source 1 LUT1/1 -> HW Delay1/1
  Source 1 LUT3/1 -> HW Delay3/1
  Source 1 LUT4/1 -> HW Delay4/1
  Source 1 LUT5/1 -> HW Delay5/1
  Delay/1 -> valid_out/1
  Source 1 LUT8/1 -> HW Delay8/1
  modTestSigSel/1 -> Multiport Switch2/1
  HW Delay/1 -> Multiport Switch2/2
  HW Delay6/1 -> Multiport Switch2/8
  HW Delay2/1 -> Multiport Switch2/4
  HW Delay7/1 -> Multiport Switch2/9
  HW Delay3/1 -> Multiport Switch2/5
  HW Delay4/1 -> Multiport Switch2/6
  HW Delay5/1 -> Multiport Switch2/7
  HW Delay9/1 -> Multiport Switch2/11
  Multiport Switch2/1 -> Data Type Conversion/1
  Data Type Conversion/1 -> data_out/1

== system gm_soc_dlmc_rfsoc_dut/FWFT_FIFO/hdl_fwft_fifo/dtci ==
  u : Inport  OutDataTypeStr=fixdt(0,32,0,'DataTypeOverride', 'Off')  SampleTime=3.90625e-09
  Conversion : DataTypeConversion  OutDataTypeStr=uint32  SaturateOnIntegerOverflow=off  RndMeth=Floor  LockScale=on
  y : Outport  SampleTime=3.90625e-09
  wires:
  Conversion/1 -> y/1
  u/1 -> Conversion/1

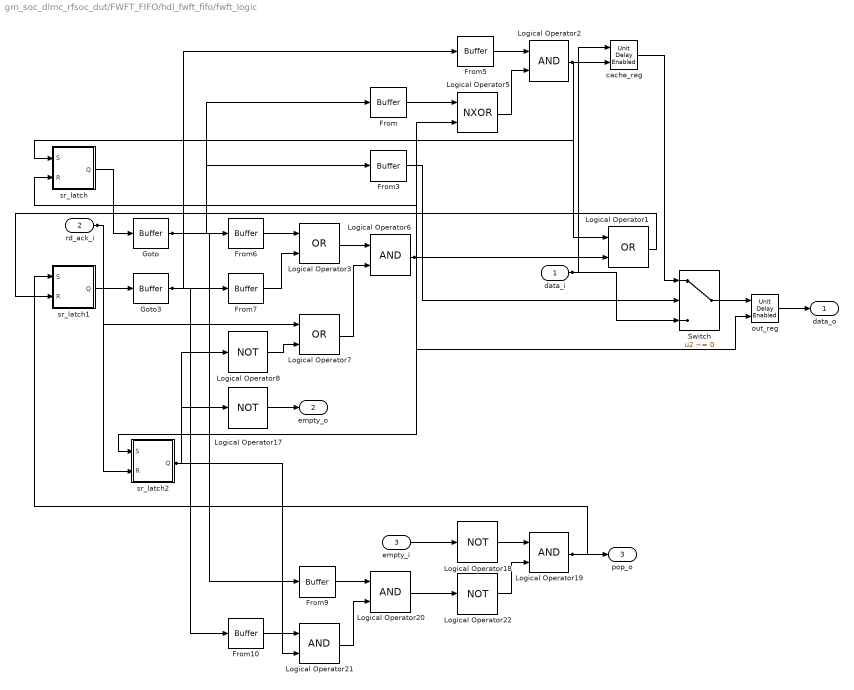
== system gm_soc_dlmc_rfsoc_dut/FWFT_FIFO/hdl_fwft_fifo/fwft_logic ==
  data_i : Inport  OutDataTypeStr=uint32  PortDimensions=1  SampleTime=3.90625e-09
  rd_ack_i : Inport  Port=2  OutDataTypeStr=boolean  PortDimensions=1  SampleTime=3.90625e-09
  empty_i : Inport  Port=3  OutDataTypeStr=boolean  PortDimensions=1  SampleTime=3.90625e-09
  From{,3,5..7,9..10} (7 alike) : hdlmdlgenlib/Buffer
  Goto : hdlmdlgenlib/Buffer
  Goto3 : hdlmdlgenlib/Buffer
  Logical Operator1 : Logic  Operator=OR  AllPortsSameDT=off  OutDataTypeStr=boolean  SampleTime=3.90625e-09
  Logical Operator{8,17..18,22} (4 alike) : Logic  Operator=NOT  Inputs=1  AllPortsSameDT=off  OutDataTypeStr=boolean  SampleTime=3.90625e-09
  Logical Operator{2,6,19..21} (5 alike) : Logic  AllPortsSameDT=off  OutDataTypeStr=boolean  SampleTime=3.90625e-09
  Logical Operator3 : Logic  Operator=OR  AllPortsSameDT=off  OutDataTypeStr=boolean  SampleTime=3.90625e-09
  Logical Operator5 : Logic  Operator=NXOR  AllPortsSameDT=off  OutDataTypeStr=boolean  SampleTime=3.90625e-09
  Logical Operator7 : Logic  Operator=OR  AllPortsSameDT=off  OutDataTypeStr=boolean  SampleTime=3.90625e-09
  Switch : Switch  Criteria=u2 ~= 0  Threshold="fi(0,0,1,0,\"hex\",\"0\")"  OutDataTypeStr=uint32  SampleTime=3.90625e-09  SaturateOnIntegerOverflow=off  InputSameDT=off
  cache_reg : simulink_need_slupdate/Unit Delay Enabled  vinit=double(0)  tsamp=-1
  out_reg : simulink_need_slupdate/Unit Delay Enabled  vinit=double(0)  tsamp=-1
  sr_latch : Subsystem
  sr_latch1 : Subsystem
  sr_latch2 : Subsystem
  data_o : Outport  SampleTime=3.90625e-09  VectorParamsAs1DForOutWhenUnconnected=off
  empty_o : Outport  Port=2  SampleTime=3.90625e-09  VectorParamsAs1DForOutWhenUnconnected=off
  pop_o : Outport  Port=3  SampleTime=3.90625e-09  VectorParamsAs1DForOutWhenUnconnected=off
  wires:
  Goto/1 -> From9/1, From3/1, From6/1, From/1
  sr_latch/1(Q) -> Goto/1
  empty_i/1 -> Logical Operator18/1
  From9/1 -> Logical Operator20/1
  From6/1 -> Logical Operator3/1
  rd_ack_i/1 -> Logical Operator7/1, sr_latch2/2(R)
  sr_latch1/1(Q) -> Goto3/1
  sr_latch2/1(Q) -> Logical Operator17/1, Logical Operator8/1, Logical Operator21/2
  Logical Operator7/1 -> Logical Operator6/2
  Goto3/1 -> From7/1, From10/1, From5/1
  From7/1 -> Logical Operator3/2
  Logical Operator8/1 -> Logical Operator7/2
  Logical Operator17/1 -> empty_o/1
  From10/1 -> Logical Operator21/1
  Logical Operator3/1 -> Logical Operator6/1
  Logical Operator6/1 -> sr_latch2/1(S), out_reg/2, Logical Operator1/2, sr_latch/2(R), Logical Operator5/2
  Logical Operator21/1 -> Logical Operator20/2
  From/1 -> Logical Operator5/1
  From3/1 -> Switch/2
  Logical Operator20/1 -> Logical Operator22/1
  From5/1 -> Logical Operator2/1
  Switch/1 -> out_reg/1
  Logical Operator5/1 -> Logical Operator2/2
  Logical Operator18/1 -> Logical Operator19/1
  Logical Operator22/1 -> Logical Operator19/2
  Logical Operator1/1 -> sr_latch1/2(R)
  Logical Operator2/1 -> sr_latch/1(S), cache_reg/2, Logical Operator1/1
  data_i/1 -> Switch/3, cache_reg/1
  Logical Operator19/1 -> sr_latch1/1(S), pop_o/1
  cache_reg/1 -> Switch/1
  out_reg/1 -> data_o/1

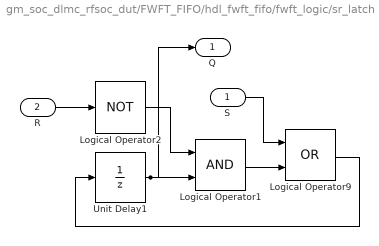
== system gm_soc_dlmc_rfsoc_dut/FWFT_FIFO/hdl_fwft_fifo/fwft_logic/sr_latch ==
  S : Inport  OutDataTypeStr=boolean  PortDimensions=1  SampleTime=3.90625e-09
  R : Inport  Port=2  OutDataTypeStr=boolean  PortDimensions=1  SampleTime=3.90625e-09
  Logical Operator1 : Logic  AllPortsSameDT=off  OutDataTypeStr=boolean  SampleTime=3.90625e-09
  Logical Operator2 : Logic  Operator=NOT  Inputs=1  AllPortsSameDT=off  OutDataTypeStr=boolean  SampleTime=3.90625e-09
  Logical Operator9 : Logic  Operator=OR  AllPortsSameDT=off  OutDataTypeStr=boolean  SampleTime=3.90625e-09
  Unit Delay1 : UnitDelay  SampleTime=3.90625e-09
  Q : Outport  SampleTime=3.90625e-09  VectorParamsAs1DForOutWhenUnconnected=off
  wires:
  R/1 -> Logical Operator2/1
  Logical Operator1/1 -> Logical Operator9/2
  Logical Operator2/1 -> Logical Operator1/1
  Logical Operator9/1 -> Unit Delay1/1
  Unit Delay1/1 -> Q/1, Logical Operator1/2
  S/1 -> Logical Operator9/1

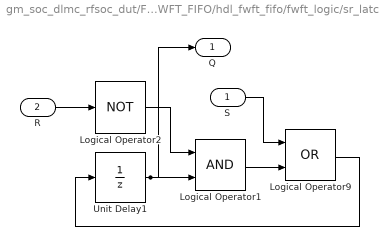
== system gm_soc_dlmc_rfsoc_dut/FWFT_FIFO/hdl_fwft_fifo/fwft_logic/sr_latch1 ==
  S : Inport  OutDataTypeStr=boolean  PortDimensions=1  SampleTime=3.90625e-09
  R : Inport  Port=2  OutDataTypeStr=boolean  PortDimensions=1  SampleTime=3.90625e-09
  Logical Operator1 : Logic  AllPortsSameDT=off  OutDataTypeStr=boolean  SampleTime=3.90625e-09
  Logical Operator2 : Logic  Operator=NOT  Inputs=1  AllPortsSameDT=off  OutDataTypeStr=boolean  SampleTime=3.90625e-09
  Logical Operator9 : Logic  Operator=OR  AllPortsSameDT=off  OutDataTypeStr=boolean  SampleTime=3.90625e-09
  Unit Delay1 : UnitDelay  SampleTime=3.90625e-09
  Q : Outport  SampleTime=3.90625e-09  VectorParamsAs1DForOutWhenUnconnected=off
  wires:
  Logical Operator1/1 -> Logical Operator9/2
  Logical Operator2/1 -> Logical Operator1/1
  R/1 -> Logical Operator2/1
  Logical Operator9/1 -> Unit Delay1/1
  Unit Delay1/1 -> Q/1, Logical Operator1/2
  S/1 -> Logical Operator9/1

== system gm_soc_dlmc_rfsoc_dut/FWFT_FIFO/hdl_fwft_fifo/fwft_logic/sr_latch2 ==
  S : Inport  OutDataTypeStr=boolean  PortDimensions=1  SampleTime=3.90625e-09
  R : Inport  Port=2  OutDataTypeStr=boolean  PortDimensions=1  SampleTime=3.90625e-09
  Logical Operator1 : Logic  AllPortsSameDT=off  OutDataTypeStr=boolean  SampleTime=3.90625e-09
  Logical Operator2 : Logic  Operator=NOT  Inputs=1  AllPortsSameDT=off  OutDataTypeStr=boolean  SampleTime=3.90625e-09
  Logical Operator9 : Logic  Operator=OR  AllPortsSameDT=off  OutDataTypeStr=boolean  SampleTime=3.90625e-09
  Unit Delay1 : UnitDelay  SampleTime=3.90625e-09
  Q : Outport  SampleTime=3.90625e-09  VectorParamsAs1DForOutWhenUnconnected=off
  wires:
  R/1 -> Logical Operator2/1
  Logical Operator1/1 -> Logical Operator9/2
  S/1 -> Logical Operator9/1
  Logical Operator2/1 -> Logical Operator1/1
  Logical Operator9/1 -> Unit Delay1/1
  Unit Delay1/1 -> Q/1, Logical Operator1/2
